simulink model "blur_control"  (R2025b)
settings: Solver=VariableStepAuto  StartTime=0.0  StopTime=100  RelTol=1e-3
libraries: fuzblock x1
settings Model: Creator=alosw  LastModifiedBy=alosw

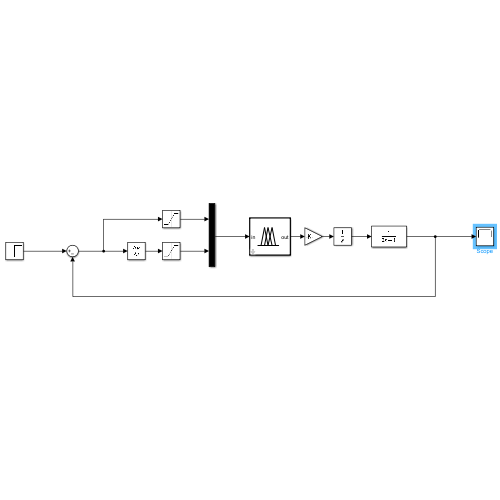
[thumbnail: Simulink's stored preview of the top-level diagram]
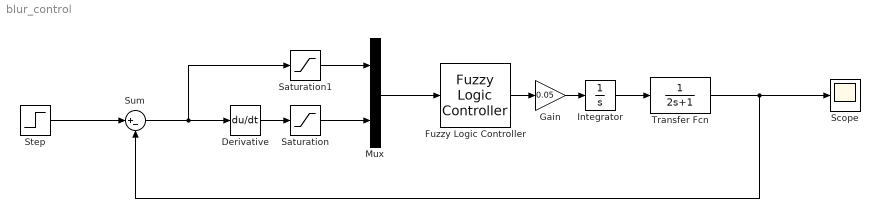
== system blur_control ==
  Derivative : Derivative
  Fuzzy Logic Controller : fuzblock/Fuzzy Logic  Controller  FIS='myFis.fis'  OutputSampleNumber=101  DataType=double  UseLookupTable=off  NumBreakpoints=10  FuzzifiedInputs=off  RuleFiringStrengths=off  RuleOutputs=off  AggregatedOutputs=off  SimulateUsing=Interpreted execution  OutOfRangeInputValueMessage=warning  NoRuleFiredMessage=warning  EmptyOutputFuzzySetMessage=warning
  Gain : Gain  Gain=0.05
  Integrator : Integrator
  Mux : Mux  Inputs=2
  Saturation : Saturate  UpperLimit=2  LowerLimit=-2
  Saturation1 : Saturate  UpperLimit=2  LowerLimit=-2
  Scope : Scope
      settings: ActiveDisplayYMinimum=-2.2006702699456442  ActiveDisplayYMaximum=3.8811599212784982
  Step : Step  SampleTime=0
  Sum : Sum  Inputs=|+-
  Transfer Fcn : TransferFcn  Denominator=[2 1]
  wires:
  Step/1 -> Sum/1
  Sum/1 -> Saturation1/1, Derivative/1
  Transfer Fcn/1 -> Sum/2, Scope/1
  Derivative/1 -> Saturation/1
  Saturation/1 -> Mux/2
  Saturation1/1 -> Mux/1
  Mux/1 -> Fuzzy Logic Controller/1
  Integrator/1 -> Transfer Fcn/1
  Fuzzy Logic Controller/1 -> Gain/1
  Gain/1 -> Integrator/1
